simulink model "GFMUPS100k_CPP"  (R2024b)
settings: Solver=ode2  StartTime=0.0  StopTime=6  FixedStep=5e-7  RelTol=1e-3
model workspace (MAT data in the model file):
  amp = 0
  f1 = 1000
undefined symbols (not defined in the file or in its folder): DiscIntNeverNeededParam, L
libraries: spsIGBTDiodeLib x12, slpidlib x12, spsabctodq0Lib x10, spsSeriesRLCBranchLib x9, spsPLL3phLib x8, spsThreePhaseSeriesRLCBranchLib x8, spsDiodeLib x6, dspstat3 x5, spsVoltageMeasurementLib x4, spsThreePhaseVIMeasurementLib x4, spsPower3phInstantaneousLib x3, spsControlledCurrentSourceLib x3
(part 3 of 4)

== system GFMUPS100k_CPP/基于自适应虚拟电流/d轴电压 ==
  presignal : Inport
  Ivd : Inport  Port=2
  MATLAB Function : MATLAB Function  TreatAsAtomicUnit=on
  PID Controller1 : slpidlib/PID Controller  Controller=PI  Form=Parallel  TimeDomain=Discrete-time  UseExternalTs=off  SampleTime=-1  IntegratorMethod=Forward Euler  FilterMethod=Forward Euler  ControllerParametersSource=internal  P=1.4  I=0.2  UseKiTs=off  D=0  UseExternalDerivativeSource=off  N=100  UseFilter=on  TunerSelectOption=Transfer Function Based (PID Tuner App)  InitialConditionSource=internal  InitialConditionForIntegrator=0  InitialConditionForFilter=0  DifferentiatorICPrevScaledInput=0  ExternalReset=none  TrackingMode=off  Kt=1  LimitOutput=off  SatLimitsSource=internal  UpperSaturationLimit=inf  LowerSaturationLimit=-inf  LinearizeAsGain=on  AntiWindupMode=none  Kb=1  LimitIntegrator=off  UpperIntegratorSaturationLimit=inf  LowerIntegratorSaturationLimit=-inf  POutMin=[]  POutMax=[]  IOutMin=[]  IOutMax=[]  DOutMin=[]  DOutMax=[]  NOutMin=[]  NOutMax=[]  SumOutMin=[]  SumOutMax=[]  SaturationOutMin=[]  SaturationOutMax=[]  PParamMin=[]  PParamMax=[]  IParamMin=[]  IParamMax=[]  DParamMin=[]  DParamMax=[]  NParamMin=[]  NParamMax=[]  KbParamMin=[]  KbParamMax=[]  KtParamMin=[]  KtParamMax=[]  KbOutMin=[]  KbOutMax=[]  KtOutMin=[]  KtOutMax=[]  IntegratorOutMin=[]  IntegratorOutMax=[]  FilterOutMin=[]  FilterOutMax=[]  SumI1OutMin=[]  SumI1OutMax=[]  SumI2OutMin=[]  SumI2OutMax=[]  SumI3OutMin=[]  SumI3OutMax=[]  SumI4OutMin=[]  SumI4OutMax=[]  SumDOutMin=[]  SumDOutMax=[]  DifferentiatorOutMin=[]  DifferentiatorOutMax=[]  FilterDiffOutCoefMin=[]  FilterDiffOutCoefMax=[]  ReciprocalOutMin=[]  ReciprocalOutMax=[]  SumDenOutMin=[]  SumDenOutMax=[]  SumNumOutMin=[]  SumNumOutMax=[]  DivideOutMin=[]  DivideOutMax=[]  UdiffTsProdOutMin=[]  UdiffTsProdOutMax=[]  NTsProdOutMin=[]  NTsProdOutMax=[]  UintegralTsProdOutMin=[]  UintegralTsProdOutMax=[]  UngainTsProdOutMin=[]  UngainTsProdOutMax=[]  ClampingZeroOutDataTypeStr=Inherit: Inherit via back propagation  ClampingZeroOutMin=[]  ClampingZeroOutMax=[]  FilterDenConstantOutDataTypeStr=Inherit: Inherit via back propagation  FilterDenConstantOutMin=[]  FilterDenConstantOutMax=[]  PCopyOutDataTypeStr=Inherit: Inherit via back propagation  PCopyOutMin=[]  PCopyOutMax=[]  NCopyOutDataTypeStr=Inherit: Inherit via back propagation  NCopyOutMin=[]  NCopyOutMax=[]  IntegratorContinuousStateAttributes=''  IntegratorStateMustResolveToSignalObject=off  IntegratorRTWStateStorageClass=Auto  FilterContinuousStateAttributes=''  FilterStateMustResolveToSignalObject=off  FilterRTWStateStorageClass=Auto  ParallelPVariant=InternalParameters  IdealPVariant=Disabled  IVariant=InternalParameters  DVariant=Disabled  IntegratorVariant=Discrete  SatVariant=Disabled  AWVariant=Passthrough  PCopyVariant=Disabled  TRVariant=Disabled  FdbkBlocksVariant=Forward  IdealPFdbkVariant=Disabled  SatFdbkVariant=Disabled  DerivativeFilterVariant=Disabled  NVariant=Disabled  NCopyVariant=Disabled_SignalSpec  FilterICVariant=Disabled  IntegratorICVariant=InternalICs  ExternalResetVariant=Disabled  TRSumVariant=Passthrough  SumFdbkVariant=Disabled  SumVariant=Sum_PI  TsampFilterVariant=InternalTs  TsampNgainVariant=Passthrough  TsampIntegralVariant=Disabled_SignalSpec  ExternalSaturationOutDataTypeStr=Inherit: Same as second input  DerivativeSourceVariant=Disabled  PreIntVariant=InternalPreInt
  "deta U " : Outport
  wires:
  MATLAB Function/1(y) -> "deta U "/1
  presignal/1 -> MATLAB Function/2(presignal)
  Ivd/1 -> PID Controller1/1
  PID Controller1/1 -> MATLAB Function/1(u)

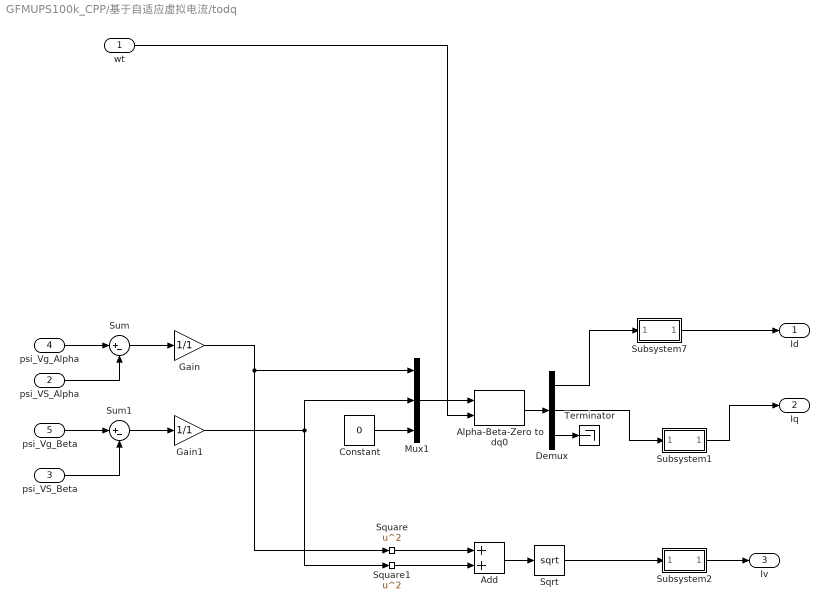
== system GFMUPS100k_CPP/基于自适应虚拟电流/todq ==
  wt : Inport
  psi_VS_Alpha : Inport  Port=2
  psi_VS_Beta : Inport  Port=3
  psi_Vg_Alpha : Inport  Port=4
  psi_Vg_Beta : Inport  Port=5
  Add : Sum
  Alpha-Beta-Zero to dq0 : spsAlphaBetaZerotodq0Lib/Alpha-Beta-Zero to dq0  Alignment=90 degrees behind phase A axis
  Constant : Constant  Value=0
  Demux : Demux  Outputs=3
  Gain : Gain  Gain=1/1
  Gain1 : Gain  Gain=1/1
  Mux1 : Mux  Inputs=3
  Sqrt : Sqrt
  Square : Math  Operator=square
  Square1 : Math  Operator=square
  Subsystem1 : Subsystem
  Subsystem2 : Subsystem
  Subsystem7 : Subsystem
  Sum : Sum  Inputs=|+-
  Sum1 : Sum  Inputs=|+-
  Terminator : Terminator
  Id : Outport
  Iq : Outport  Port=2
  Iv : Outport  Port=3
  wires:
  Demux/2 -> Subsystem1/1(In1)
  Constant/1 -> Mux1/3
  Square/1 -> Add/1
  Add/1 -> Sqrt/1
  Mux1/1 -> Alpha-Beta-Zero to dq0/1
  Square1/1 -> Add/2
  Demux/1 -> Subsystem7/1(In1)
  Gain/1 -> Square/1, Mux1/1
  Sqrt/1 -> Subsystem2/1(In1)
  Demux/3 -> Terminator/1
  Sum1/1 -> Gain1/1
  wt/1 -> Alpha-Beta-Zero to dq0/2
  Sum/1 -> Gain/1
  Alpha-Beta-Zero to dq0/1 -> Demux/1
  Gain1/1 -> Mux1/2, Square1/1
  psi_VS_Beta/1 -> Sum1/2
  psi_Vg_Beta/1 -> Sum1/1
  psi_Vg_Alpha/1 -> Sum/1
  psi_VS_Alpha/1 -> Sum/2
  Subsystem7/1(Out1) -> Id/1
  Subsystem1/1(Out1) -> Iq/1
  Subsystem2/1(Out1) -> Iv/1

== system GFMUPS100k_CPP/基于自适应虚拟电流/标幺 ==
  abc : Inport
  abc1 : Inport  Port=2
  Demux : Demux  Outputs=3
  Demux1 : Demux  Outputs=3
  Gain1 : Gain  Gain=1/311
  Gain2 : Gain  Gain=1/311
  Scope1 : Scope
  Terminator1 : Terminator
  Terminator2 : Terminator
  abc to Alpha-Beta-Zero1 : spsabctoAlphaBetaZeroLib/abc to Alpha-Beta-Zero
  abc to Alpha-Beta-Zero2 : spsabctoAlphaBetaZeroLib/abc to Alpha-Beta-Zero
  Vs_alpha : Outport
  Vs_beta : Outport  Port=2
  Vg_alpha1 : Outport  Port=3
  Vg_beta1 : Outport  Port=4
  wires:
  Demux1/2 -> Vg_beta1/1
  Demux1/3 -> Terminator2/1
  Demux1/1 -> Vg_alpha1/1
  Demux/2 -> Vs_beta/1
  abc to Alpha-Beta-Zero2/1 -> Demux1/1
  abc1/1 -> Gain1/1
  abc to Alpha-Beta-Zero1/1 -> Demux/1
  Demux/3 -> Terminator1/1
  Gain2/1 -> abc to Alpha-Beta-Zero1/1
  Demux/1 -> Vs_alpha/1
  abc/1 -> Gain2/1
  Gain1/1 -> Scope1/1, abc to Alpha-Beta-Zero2/1

== system GFMUPS100k_CPP/基于自适应虚拟电流/自适应PI ==
  Ivq_re : Inport
  Kp_base : Inport  Port=2
  Ki_base : Inport  Port=3
  Gain : Gain
  PID Controller : slpidlib/PID Controller  Controller=PI  Form=Parallel  TimeDomain=Discrete-time  UseExternalTs=off  SampleTime=5e-05  IntegratorMethod=Forward Euler  FilterMethod=Forward Euler  ControllerParametersSource=external  P=1  I=1  UseKiTs=off  D=0  UseExternalDerivativeSource=off  N=100  UseFilter=on  TunerSelectOption=Transfer Function Based (PID Tuner App)  InitialConditionSource=internal  InitialConditionForIntegrator=0  InitialConditionForFilter=0  DifferentiatorICPrevScaledInput=0  ExternalReset=none  TrackingMode=off  Kt=1  LimitOutput=off  SatLimitsSource=internal  UpperSaturationLimit=inf  LowerSaturationLimit=-inf  LinearizeAsGain=on  AntiWindupMode=none  Kb=1  LimitIntegrator=off  UpperIntegratorSaturationLimit=inf  LowerIntegratorSaturationLimit=-inf  POutMin=[]  POutMax=[]  IOutMin=[]  IOutMax=[]  DOutMin=[]  DOutMax=[]  NOutMin=[]  NOutMax=[]  SumOutMin=[]  SumOutMax=[]  SaturationOutMin=[]  SaturationOutMax=[]  PParamMin=[]  PParamMax=[]  IParamMin=[]  IParamMax=[]  DParamMin=[]  DParamMax=[]  NParamMin=[]  NParamMax=[]  KbParamMin=[]  KbParamMax=[]  KtParamMin=[]  KtParamMax=[]  KbOutMin=[]  KbOutMax=[]  KtOutMin=[]  KtOutMax=[]  IntegratorOutMin=[]  IntegratorOutMax=[]  FilterOutMin=[]  FilterOutMax=[]  SumI1OutMin=[]  SumI1OutMax=[]  SumI2OutMin=[]  SumI2OutMax=[]  SumI3OutMin=[]  SumI3OutMax=[]  SumI4OutMin=[]  SumI4OutMax=[]  SumDOutMin=[]  SumDOutMax=[]  DifferentiatorOutMin=[]  DifferentiatorOutMax=[]  FilterDiffOutCoefMin=[]  FilterDiffOutCoefMax=[]  ReciprocalOutMin=[]  ReciprocalOutMax=[]  SumDenOutMin=[]  SumDenOutMax=[]  SumNumOutMin=[]  SumNumOutMax=[]  DivideOutMin=[]  DivideOutMax=[]  UdiffTsProdOutMin=[]  UdiffTsProdOutMax=[]  NTsProdOutMin=[]  NTsProdOutMax=[]  UintegralTsProdOutMin=[]  UintegralTsProdOutMax=[]  UngainTsProdOutMin=[]  UngainTsProdOutMax=[]  ClampingZeroOutDataTypeStr=Inherit: Inherit via back propagation  ClampingZeroOutMin=[]  ClampingZeroOutMax=[]  FilterDenConstantOutDataTypeStr=Inherit: Inherit via back propagation  FilterDenConstantOutMin=[]  FilterDenConstantOutMax=[]  PCopyOutDataTypeStr=Inherit: Inherit via back propagation  PCopyOutMin=[]  PCopyOutMax=[]  NCopyOutDataTypeStr=Inherit: Inherit via back propagation  NCopyOutMin=[]  NCopyOutMax=[]  IntegratorContinuousStateAttributes=''  IntegratorStateMustResolveToSignalObject=off  IntegratorRTWStateStorageClass=Auto  FilterContinuousStateAttributes=''  FilterStateMustResolveToSignalObject=off  FilterRTWStateStorageClass=Auto  ParallelPVariant=ExternalParameters  IdealPVariant=Disabled  IVariant=ExternalParameters  DVariant=Disabled  IntegratorVariant=Discrete  SatVariant=Disabled  AWVariant=Passthrough  PCopyVariant=Disabled  TRVariant=Disabled  FdbkBlocksVariant=Forward  IdealPFdbkVariant=Disabled  SatFdbkVariant=Disabled  DerivativeFilterVariant=Disabled  NVariant=Disabled  NCopyVariant=Disabled_SignalSpec  FilterICVariant=Disabled  IntegratorICVariant=InternalICs  ExternalResetVariant=Disabled  TRSumVariant=Passthrough  SumFdbkVariant=Disabled  SumVariant=Sum_PI  TsampFilterVariant=InternalTs  TsampNgainVariant=Passthrough  TsampIntegralVariant=Disabled_SignalSpec  ExternalSaturationOutDataTypeStr=Inherit: Same as second input  DerivativeSourceVariant=Disabled  PreIntVariant=InternalPreInt
  Scope1 : Scope  NumInputPorts=2
  adaptive_PI : MATLAB Function  TreatAsAtomicUnit=on  SystemSampleTime=5e-05
  预同步 : Subsystem
  预同步1 : Subsystem
  Out1 : Outport
  wires:
  Ki_base/1 -> adaptive_PI/3(Ki_base)
  Ivq_re/1 -> adaptive_PI/1(Ivq_re), PID Controller/1
  adaptive_PI/1(Kp_act) -> 预同步/1(d_theta)
  Kp_base/1 -> adaptive_PI/2(Kp_base)
  adaptive_PI/2(Ki_act) -> 预同步1/1(d_theta)
  Gain/1 -> Out1/1
  PID Controller/1 -> Gain/1
  预同步/1(Out1) -> PID Controller/2, Scope1/1
  预同步1/1(Out1) -> PID Controller/3, Scope1/2

== system GFMUPS100k_CPP/基于转dq的预同步控制1/电压预同步 ==
  Vg : Inport
  Vabc : Inport  Port=2
  presignal : Inport  Port=3
  Constant1 : Constant  Value=0
  PID Controller2 : slpidlib/PID Controller  Controller=PI  Form=Parallel  TimeDomain=Discrete-time  UseExternalTs=off  SampleTime=5e-05  IntegratorMethod=Forward Euler  FilterMethod=Forward Euler  ControllerParametersSource=internal  P=0.8  I=0  UseKiTs=off  D=0  UseExternalDerivativeSource=off  N=100  UseFilter=on  TunerSelectOption=Transfer Function Based (PID Tuner App)  InitialConditionSource=internal  InitialConditionForIntegrator=0  InitialConditionForFilter=0  DifferentiatorICPrevScaledInput=0  ExternalReset=none  TrackingMode=off  Kt=1  LimitOutput=off  SatLimitsSource=internal  UpperSaturationLimit=inf  LowerSaturationLimit=-inf  LinearizeAsGain=on  AntiWindupMode=none  Kb=1  LimitIntegrator=off  UpperIntegratorSaturationLimit=inf  LowerIntegratorSaturationLimit=-inf  POutMin=[]  POutMax=[]  IOutMin=[]  IOutMax=[]  DOutMin=[]  DOutMax=[]  NOutMin=[]  NOutMax=[]  SumOutMin=[]  SumOutMax=[]  SaturationOutMin=[]  SaturationOutMax=[]  PParamMin=[]  PParamMax=[]  IParamMin=[]  IParamMax=[]  DParamMin=[]  DParamMax=[]  NParamMin=[]  NParamMax=[]  KbParamMin=[]  KbParamMax=[]  KtParamMin=[]  KtParamMax=[]  KbOutMin=[]  KbOutMax=[]  KtOutMin=[]  KtOutMax=[]  IntegratorOutMin=[]  IntegratorOutMax=[]  FilterOutMin=[]  FilterOutMax=[]  SumI1OutMin=[]  SumI1OutMax=[]  SumI2OutMin=[]  SumI2OutMax=[]  SumI3OutMin=[]  SumI3OutMax=[]  SumI4OutMin=[]  SumI4OutMax=[]  SumDOutMin=[]  SumDOutMax=[]  DifferentiatorOutMin=[]  DifferentiatorOutMax=[]  FilterDiffOutCoefMin=[]  FilterDiffOutCoefMax=[]  ReciprocalOutMin=[]  ReciprocalOutMax=[]  SumDenOutMin=[]  SumDenOutMax=[]  SumNumOutMin=[]  SumNumOutMax=[]  DivideOutMin=[]  DivideOutMax=[]  UdiffTsProdOutMin=[]  UdiffTsProdOutMax=[]  NTsProdOutMin=[]  NTsProdOutMax=[]  UintegralTsProdOutMin=[]  UintegralTsProdOutMax=[]  UngainTsProdOutMin=[]  UngainTsProdOutMax=[]  ClampingZeroOutDataTypeStr=Inherit: Inherit via back propagation  ClampingZeroOutMin=[]  ClampingZeroOutMax=[]  FilterDenConstantOutDataTypeStr=Inherit: Inherit via back propagation  FilterDenConstantOutMin=[]  FilterDenConstantOutMax=[]  PCopyOutDataTypeStr=Inherit: Inherit via back propagation  PCopyOutMin=[]  PCopyOutMax=[]  NCopyOutDataTypeStr=Inherit: Inherit via back propagation  NCopyOutMin=[]  NCopyOutMax=[]  IntegratorContinuousStateAttributes=''  IntegratorStateMustResolveToSignalObject=off  IntegratorRTWStateStorageClass=Auto  FilterContinuousStateAttributes=''  FilterStateMustResolveToSignalObject=off  FilterRTWStateStorageClass=Auto  ParallelPVariant=InternalParameters  IdealPVariant=Disabled  IVariant=InternalParameters  DVariant=Disabled  IntegratorVariant=Discrete  SatVariant=Disabled  AWVariant=Passthrough  PCopyVariant=Disabled  TRVariant=Disabled  FdbkBlocksVariant=Forward  IdealPFdbkVariant=Disabled  SatFdbkVariant=Disabled  DerivativeFilterVariant=Disabled  NVariant=Disabled  NCopyVariant=Disabled_SignalSpec  FilterICVariant=Disabled  IntegratorICVariant=InternalICs  ExternalResetVariant=Disabled  TRSumVariant=Passthrough  SumFdbkVariant=Disabled  SumVariant=Sum_PI  TsampFilterVariant=InternalTs  TsampNgainVariant=Passthrough  TsampIntegralVariant=Disabled_SignalSpec  ExternalSaturationOutDataTypeStr=Inherit: Same as second input  DerivativeSourceVariant=Disabled  PreIntVariant=InternalPreInt
  RMS1 : dspstat3/RMS  run=off  directionMode=Each column  dimension=1  InputProcessing=Columns as channels (frame based)  reset_popup=None
  RMS2 : dspstat3/RMS  run=off  directionMode=Each column  dimension=1  InputProcessing=Columns as channels (frame based)  reset_popup=None
  Scope : Scope
  Sum4 : Sum  Inputs=|+-
  Switch : Switch  Criteria=u2 > Threshold  SaturateOnIntegerOverflow=off  InputSameDT=off
  d_U : Outport
  wires:
  presignal/1 -> Switch/2
  Constant1/1 -> Switch/3
  PID Controller2/1 -> Switch/1
  Sum4/1 -> Scope/1, PID Controller2/1
  Switch/1 -> d_U/1
  Vg/1 -> RMS2/1
  Vabc/1 -> RMS1/1
  RMS2/1 -> Sum4/1
  RMS1/1 -> Sum4/2

== system GFMUPS100k_CPP/基于转dq的预同步控制1/相位预同步 ==
  Vg : Inport
  Vabc : Inport  Port=2
  presignal : Inport  Port=3
  Constant5 : Constant  Value=0
  Demux : Demux  Outputs=3
  Gain : Gain  Gain=-1
  PID Controller1 : slpidlib/PID Controller  Controller=PI  Form=Parallel  TimeDomain=Discrete-time  UseExternalTs=off  SampleTime=5e-05  IntegratorMethod=Forward Euler  FilterMethod=Forward Euler  ControllerParametersSource=internal  P=0.4  I=0.01  UseKiTs=off  D=0  UseExternalDerivativeSource=off  N=100  UseFilter=on  TunerSelectOption=Transfer Function Based (PID Tuner App)  InitialConditionSource=internal  InitialConditionForIntegrator=0  InitialConditionForFilter=0  DifferentiatorICPrevScaledInput=0  ExternalReset=none  TrackingMode=off  Kt=1  LimitOutput=off  SatLimitsSource=internal  UpperSaturationLimit=inf  LowerSaturationLimit=-inf  LinearizeAsGain=on  AntiWindupMode=none  Kb=1  LimitIntegrator=off  UpperIntegratorSaturationLimit=inf  LowerIntegratorSaturationLimit=-inf  POutMin=[]  POutMax=[]  IOutMin=[]  IOutMax=[]  DOutMin=[]  DOutMax=[]  NOutMin=[]  NOutMax=[]  SumOutMin=[]  SumOutMax=[]  SaturationOutMin=[]  SaturationOutMax=[]  PParamMin=[]  PParamMax=[]  IParamMin=[]  IParamMax=[]  DParamMin=[]  DParamMax=[]  NParamMin=[]  NParamMax=[]  KbParamMin=[]  KbParamMax=[]  KtParamMin=[]  KtParamMax=[]  KbOutMin=[]  KbOutMax=[]  KtOutMin=[]  KtOutMax=[]  IntegratorOutMin=[]  IntegratorOutMax=[]  FilterOutMin=[]  FilterOutMax=[]  SumI1OutMin=[]  SumI1OutMax=[]  SumI2OutMin=[]  SumI2OutMax=[]  SumI3OutMin=[]  SumI3OutMax=[]  SumI4OutMin=[]  SumI4OutMax=[]  SumDOutMin=[]  SumDOutMax=[]  DifferentiatorOutMin=[]  DifferentiatorOutMax=[]  FilterDiffOutCoefMin=[]  FilterDiffOutCoefMax=[]  ReciprocalOutMin=[]  ReciprocalOutMax=[]  SumDenOutMin=[]  SumDenOutMax=[]  SumNumOutMin=[]  SumNumOutMax=[]  DivideOutMin=[]  DivideOutMax=[]  UdiffTsProdOutMin=[]  UdiffTsProdOutMax=[]  NTsProdOutMin=[]  NTsProdOutMax=[]  UintegralTsProdOutMin=[]  UintegralTsProdOutMax=[]  UngainTsProdOutMin=[]  UngainTsProdOutMax=[]  ClampingZeroOutDataTypeStr=Inherit: Inherit via back propagation  ClampingZeroOutMin=[]  ClampingZeroOutMax=[]  FilterDenConstantOutDataTypeStr=Inherit: Inherit via back propagation  FilterDenConstantOutMin=[]  FilterDenConstantOutMax=[]  PCopyOutDataTypeStr=Inherit: Inherit via back propagation  PCopyOutMin=[]  PCopyOutMax=[]  NCopyOutDataTypeStr=Inherit: Inherit via back propagation  NCopyOutMin=[]  NCopyOutMax=[]  IntegratorContinuousStateAttributes=''  IntegratorStateMustResolveToSignalObject=off  IntegratorRTWStateStorageClass=Auto  FilterContinuousStateAttributes=''  FilterStateMustResolveToSignalObject=off  FilterRTWStateStorageClass=Auto  ParallelPVariant=InternalParameters  IdealPVariant=Disabled  IVariant=InternalParameters  DVariant=Disabled  IntegratorVariant=Discrete  SatVariant=Disabled  AWVariant=Passthrough  PCopyVariant=Disabled  TRVariant=Disabled  FdbkBlocksVariant=Forward  IdealPFdbkVariant=Disabled  SatFdbkVariant=Disabled  DerivativeFilterVariant=Disabled  NVariant=Disabled  NCopyVariant=Disabled_SignalSpec  FilterICVariant=Disabled  IntegratorICVariant=InternalICs  ExternalResetVariant=Disabled  TRSumVariant=Passthrough  SumFdbkVariant=Disabled  SumVariant=Sum_PI  TsampFilterVariant=InternalTs  TsampNgainVariant=Passthrough  TsampIntegralVariant=Disabled_SignalSpec  ExternalSaturationOutDataTypeStr=Inherit: Same as second input  DerivativeSourceVariant=Disabled  PreIntVariant=InternalPreInt
  PLL (3ph) : spsPLL3phLib/PLL (3ph)  Fmin=45  Par_Init=[0, 60]  ParK=[180, 3200, 1]  TcD=1e-4  MaxRateChangeFreq=12  FilterCutOffFreq=25  Ts=0  AGC=on
  Scope : Scope
  Scope1 : Scope
  Switch : Switch  Criteria=u2 > Threshold  SaturateOnIntegerOverflow=off  InputSameDT=off
  Terminator : Terminator
  Terminator1 : Terminator
  Terminator2 : Terminator
  abc to dq0 : spsabctodq0Lib/abc to dq0  Alignment=90 degrees behind phase A axis
  c_theta : Outport
  wires:
  Constant5/1 -> Switch/3
  PID Controller1/1 -> Switch/1
  Switch/1 -> Scope1/1, c_theta/1
  presignal/1 -> Switch/2
  Vg/1 -> PLL (3ph)/1
  Vabc/1 -> abc to dq0/1
  abc to dq0/1 -> Demux/1
  PLL (3ph)/2 -> abc to dq0/2
  PLL (3ph)/1 -> Terminator/1
  Demux/3 -> Terminator2/1
  Demux/1 -> Terminator1/1
  Demux/2 -> Gain/1
  Gain/1 -> Scope/1, PID Controller1/1

== system GFMUPS100k_CPP/相角差计算/Subsystem1 ==
  abc : Inport
  abc1 : Inport  Port=2
  Add : Sum  Inputs=+-
  PLL (3ph)1 : spsPLL3phLib/PLL (3ph)  Fmin=45  Par_Init=[0, 60]  ParK=[180, 3200, 1]  TcD=1e-4  MaxRateChangeFreq=12  FilterCutOffFreq=25  Ts=0  AGC=on
  PLL (3ph)2 : spsPLL3phLib/PLL (3ph)  Fmin=45  Par_Init=[0, 60]  ParK=[180, 3200, 1]  TcD=1e-4  MaxRateChangeFreq=12  FilterCutOffFreq=25  Ts=0  AGC=on
  Terminator8 : Terminator
  Terminator9 : Terminator
  Out1 : Outport
  wires:
  PLL (3ph)1/1 -> Terminator9/1
  PLL (3ph)2/2 -> Add/1
  PLL (3ph)2/1 -> Terminator8/1
  PLL (3ph)1/2 -> Add/2
  Add/1 -> Out1/1
  abc/1 -> PLL (3ph)2/1
  abc1/1 -> PLL (3ph)1/1

== system GFMUPS100k_CPP/相角差计算/Subsystem2 ==
  In1 : Inport
  Add : Sum  Inputs=+-
  Add4 : Sum
  Constant : Constant  Value=2*pi
  Constant1 : Constant  Value=pi
  Constant2 : Constant  Value=pi
  Mod : Math  Operator=mod
  dete_theta : Outport
  wires:
  In1/1 -> Add4/1
  Constant1/1 -> Add/2
  Add4/1 -> Mod/1
  Constant/1 -> Mod/2
  Mod/1 -> Add/1
  Constant2/1 -> Add4/2
  Add/1 -> dete_theta/1

== system GFMUPS100k_CPP/VSG_Control/无功控制环1/Subsystem1 ==
  In1 : Inport
  Discrete-Time Integrator : DiscreteIntegrator  SampleTime=1/20000  ICPrevOutput=DiscIntNeverNeededParam  ICPrevScaledInput=DiscIntNeverNeededParam
  Gain1 : Gain  Gain=2*pi*50
  Gain2 : Gain
  Sum3 : Sum  Inputs=|+-
  Out1 : Outport
  wires:
  Sum3/1 -> Gain1/1
  Gain1/1 -> Discrete-Time Integrator/1
  Gain2/1 -> Sum3/2
  In1/1 -> Sum3/1
  Discrete-Time Integrator/1 -> Gain2/1, Out1/1

== system GFMUPS100k_CPP/VSG_Control/无功控制环1/Subsystem2 ==
  In1 : Inport
  Discrete-Time Integrator : DiscreteIntegrator  SampleTime=1/20000  ICPrevOutput=DiscIntNeverNeededParam  ICPrevScaledInput=DiscIntNeverNeededParam
  Gain1 : Gain  Gain=2*pi*50
  Gain2 : Gain
  Sum3 : Sum  Inputs=|+-
  Out1 : Outport
  wires:
  Discrete-Time Integrator/1 -> Out1/1, Gain2/1
  In1/1 -> Sum3/1
  Gain2/1 -> Sum3/2
  Gain1/1 -> Discrete-Time Integrator/1
  Sum3/1 -> Gain1/1

== system GFMUPS100k_CPP/VSG_Control/有功控制环/预同步 ==
  d_theta : Inport
  Discrete-Time Integrator : DiscreteIntegrator  SampleTime=5e-05  ICPrevOutput=DiscIntNeverNeededParam  ICPrevScaledInput=DiscIntNeverNeededParam
  Gain1 : Gain  Gain=1/0.03
  Gain2 : Gain
  Saturation : Saturate  Commented=on  UpperLimit=401.23  LowerLimit=-9.54
  Scope : Scope  NumInputPorts=2
  Sum3 : Sum  Inputs=|+-
  Out1 : Outport
  wires:
  Discrete-Time Integrator/1 -> Scope/2, Out1/1, Gain2/1
  Gain1/1 -> Discrete-Time Integrator/1
  Sum3/1 -> Gain1/1
  Gain2/1 -> Sum3/2
  d_theta/1 -> Scope/1, Sum3/1

== system GFMUPS100k_CPP/VSG_Control/虚拟阻抗（scr补偿）/Subsystem1 ==
  In1 : Inport
  Discrete-Time Integrator : DiscreteIntegrator  SampleTime=1/20000  ICPrevOutput=DiscIntNeverNeededParam  ICPrevScaledInput=DiscIntNeverNeededParam
  Gain1 : Gain  Gain=2*pi*500
  Gain2 : Gain
  Sum3 : Sum  Inputs=|+-
  Out1 : Outport
  wires:
  Discrete-Time Integrator/1 -> Out1/1, Gain2/1
  In1/1 -> Sum3/1
  Gain2/1 -> Sum3/2
  Gain1/1 -> Discrete-Time Integrator/1
  Sum3/1 -> Gain1/1

== system GFMUPS100k_CPP/VSG_Control/虚拟阻抗（scr补偿）/Subsystem7 ==
  In1 : Inport
  Discrete-Time Integrator : DiscreteIntegrator  SampleTime=1/20000  ICPrevOutput=DiscIntNeverNeededParam  ICPrevScaledInput=DiscIntNeverNeededParam
  Gain1 : Gain  Gain=2*pi*500
  Gain2 : Gain
  Sum3 : Sum  Inputs=|+-
  Out1 : Outport
  wires:
  Sum3/1 -> Gain1/1
  Gain1/1 -> Discrete-Time Integrator/1
  Gain2/1 -> Sum3/2
  In1/1 -> Sum3/1
  Discrete-Time Integrator/1 -> Gain2/1, Out1/1

== system GFMUPS100k_CPP/基于自适应虚拟电流/todq/Subsystem1 ==
  In1 : Inport
  Discrete-Time Integrator : DiscreteIntegrator  SampleTime=1/20000  ICPrevOutput=DiscIntNeverNeededParam  ICPrevScaledInput=DiscIntNeverNeededParam
  Gain1 : Gain  Gain=2*pi*50
  Gain2 : Gain
  Sum3 : Sum  Inputs=|+-
  Out1 : Outport
  wires:
  Discrete-Time Integrator/1 -> Out1/1, Gain2/1
  In1/1 -> Sum3/1
  Gain2/1 -> Sum3/2
  Gain1/1 -> Discrete-Time Integrator/1
  Sum3/1 -> Gain1/1

== system GFMUPS100k_CPP/基于自适应虚拟电流/todq/Subsystem2 ==
  In1 : Inport
  Discrete-Time Integrator : DiscreteIntegrator  SampleTime=1/20000  ICPrevOutput=DiscIntNeverNeededParam  ICPrevScaledInput=DiscIntNeverNeededParam
  Gain1 : Gain  Gain=2*pi*50
  Gain2 : Gain
  Sum3 : Sum  Inputs=|+-
  Out1 : Outport
  wires:
  Sum3/1 -> Gain1/1
  Gain1/1 -> Discrete-Time Integrator/1
  Gain2/1 -> Sum3/2
  In1/1 -> Sum3/1
  Discrete-Time Integrator/1 -> Gain2/1, Out1/1

== system GFMUPS100k_CPP/基于自适应虚拟电流/todq/Subsystem7 ==
  In1 : Inport
  Discrete-Time Integrator : DiscreteIntegrator  SampleTime=1/20000  ICPrevOutput=DiscIntNeverNeededParam  ICPrevScaledInput=DiscIntNeverNeededParam
  Gain1 : Gain  Gain=2*pi*50
  Gain2 : Gain
  Sum3 : Sum  Inputs=|+-
  Out1 : Outport
  wires:
  Sum3/1 -> Gain1/1
  Gain1/1 -> Discrete-Time Integrator/1
  Gain2/1 -> Sum3/2
  In1/1 -> Sum3/1
  Discrete-Time Integrator/1 -> Gain2/1, Out1/1

== system GFMUPS100k_CPP/基于自适应虚拟电流/自适应PI/预同步 ==
  d_theta : Inport
  Discrete-Time Integrator : DiscreteIntegrator  SampleTime=5e-05  ICPrevOutput=DiscIntNeverNeededParam  ICPrevScaledInput=DiscIntNeverNeededParam
  Gain1 : Gain  Gain=1/0.03
  Gain2 : Gain
  Saturation : Saturate  Commented=on  UpperLimit=401.23  LowerLimit=-9.54
  Sum3 : Sum  Inputs=|+-
  Out1 : Outport
  wires:
  Discrete-Time Integrator/1 -> Out1/1, Gain2/1
  Gain1/1 -> Discrete-Time Integrator/1
  Sum3/1 -> Gain1/1
  Gain2/1 -> Sum3/2
  d_theta/1 -> Sum3/1

== system GFMUPS100k_CPP/基于自适应虚拟电流/自适应PI/预同步1 ==
  d_theta : Inport
  Discrete-Time Integrator : DiscreteIntegrator  SampleTime=5e-05  ICPrevOutput=DiscIntNeverNeededParam  ICPrevScaledInput=DiscIntNeverNeededParam
  Gain1 : Gain  Gain=1/0.03
  Gain2 : Gain
  Saturation : Saturate  Commented=on  UpperLimit=401.23  LowerLimit=-9.54
  Sum3 : Sum  Inputs=|+-
  Out1 : Outport
  wires:
  d_theta/1 -> Sum3/1
  Gain2/1 -> Sum3/2
  Sum3/1 -> Gain1/1
  Gain1/1 -> Discrete-Time Integrator/1
  Discrete-Time Integrator/1 -> Gain2/1, Out1/1

== matlab function GFMUPS100k_CPP/SVPWM调制/SVPWM/第一大扇区羊角波分配 ==
  data: n input; T1 input; T2 input; T3 input; t11 output; t21 output; t31 output
function [t11,t21,t31] = vectorshare(n,T1,T2,T3)
t11=0;
t21=0;
t31=0;
if(n==1)
    t11=T1/2;
    t21=-T1/2;
    t31=-T1/2-T2;
end
if(n==2)
    t11=T1/2+T3;
    t21=T1/2;
    t31=-T1/2;
end
if(n==3)
    t11=T1/2+T3;
    t21=-T1/2;
    t31=-T1/2-T2-T3;
end
if(n==4)
    t11=T1/2+T2+T3;
    t21=T1/2;
    t31=-T1/2-T2;
end
if(n==5)
    t11=T1/2+T2+T3;
    t21=-T1/2-T2;
    t31=-T1/2-T2-T3;
end
if(n==6)
    t11=T1/2+T2+T3;
    t21=T1/2+T3;
    t31=-T1/2-T2-T3;
end

== matlab function GFMUPS100k_CPP/SVPWM调制/SVPWM/第二大扇区羊角波分配 ==
  data: n input; T1 input; T2 input; T3 input; t11 output; t21 output; t31 output
function [t11,t21,t31] = switchshare(n,T1,T2,T3)
t11=0;
t21=0;
t31=0;
if(n==1)
    t11=T1/2;
    t21=T1/2+T3;
    t31=-T1/2;
end
if(n==2)
    t11=-T1/2;
    t21=T1/2;
    t31=-T1/2-T2;
end
if(n==3)
    t11=T1/2;
    t21=T1/2+T2+T3;
    t31=-T1/2-T2;
end
if(n==4)
    t11=-T1/2;
    t21=T1/2+T3;
    t31=-T1/2-T2-T3;
end
if(n==5)
    t11=T1/2+T3;
    t21=T1/2+T2+T3;
    t31=-T1/2-T2-T3;
end
if(n==6)
    t11=-T1/2-T2;
    t21=T1/2+T3+T2;
    t31=-T1/2-T2-T3;
end

== matlab function GFMUPS100k_CPP/SVPWM调制/SVPWM/羊角波生成 ==
  data: N input; t11 input; t12 input; t13 input; YJA output; YJB output; YJC output; t21 input; t22 input; t23 input
function [YJA,YJB,YJC] = vectorshare(N,t11,t12,t13,t21,t22,t23)
YJA=0;
YJB=0;
YJC=0;
if(N==1)
    YJA=t11;
    YJB=t12;
    YJC=t13;
end
if(N==2)
    YJA=t21;
    YJB=t22;
    YJC=t23;
end
if(N==3)
    YJA=t13;
    YJB=t11;
    YJC=t12;
end
if(N==4)
    YJA=t23;
    YJB=t21;
    YJC=t22;
end
if(N==5)
    YJA=t12;
    YJB=t13;
    YJC=t11;
end
if(N==6)
    YJA=t22;
    YJB=t23;
    YJC=t21;
end

== matlab function GFMUPS100k_CPP/基于自适应虚拟电流/MATLAB Function ==
  data: u input; y output; presignal input
function y = fcn(u, presignal)
    % 如果 presignal 大于 0，输出 y 等于 u
    % 否则输出 y 等于 0
    if presignal > 0
        y = u;
    else
        y = 0;
    end
end

== matlab function GFMUPS100k_CPP/基于自适应虚拟电流/d轴电压/MATLAB Function ==
  data: u input; y output; presignal input
function y = fcn(u, presignal)
    % 如果 presignal 大于 0，输出 y 等于 u
    % 否则输出 y 等于 0
    if presignal > 0
        y = u;
    else
        y = 0;
    end
end

== matlab function GFMUPS100k_CPP/Grid_Impedance_Estimator/Positive_Sequence ==
  data: vabc input; E output; iuabc input; ilabc input; t input; reset input; source input; Vg output; theta output; Pu output; Qu output; PL output; QL output; ready output
function [E,Vg,theta,Pu,Qu,PL,QL,ready] = positive_sequence_inputs(vabc,iuabc,ilabc,t,reset,source)
%#codegen
% 200 samples at 100 us = one 50-Hz cycle, fixed-size positive sequence DFT.
% source = [line-line RMS volts, Hz, phase A sine angle in degrees].
persistent buffer sums index count
if isempty(count)   %200个采样点， 采样周期为1e-4，200*Ts，刚好是一个完整的50HZ周期  Sum保存200个点的累加  count表示收集了多少有效采样点
    buffer = zeros(6,200); sums = zeros(6,1); index = 1; count = 0;
end
if reset ~= 0
    buffer(:) = 0; sums(:) = 0; index = 1; count = 0;
end
E=0; Vg=source(1)*sqrt(2/3); theta=0;
Pu=0; Qu=0; PL=0; QL=0; ready=false;
if ~all(isfinite([vabc(:);iuabc(:);ilabc(:);t]))  %检查是不是所有输入都是正常有限数值
    buffer(:)=0; sums(:)=0; index=1; count=0;
    return
end
phi = 2*pi*source(2)*t + source(3)*pi/180-pi/2;  %电网参考角
c=cos(phi); s=sin(phi);
va=(2*vabc(1)-vabc(2)-vabc(3))/3;%abc转到β轴
vb=(vabc(2)-vabc(3))/sqrt(3);
ua=(2*iuabc(1)-iuabc(2)-iuabc(3))/3;
ub=(iuabc(2)-iuabc(3))/sqrt(3);
la=(2*ilabc(1)-ilabc(2)-ilabc(3))/3;
lb=(ilabc(2)-ilabc(3))/sqrt(3);
sample=[va*c+vb*s;vb*c-va*s;ua*c+ub*s;ub*c-ua*s;la*c+lb*s;lb*c-la*s];
sums=sums-buffer(:,index)+sample;%把200个点中旧的数据删除，加入新的数据
buffer(:,index)=sample;
index=index+1;
if index>200, index=1; end
count=min(count+1,200);
v=sums/200;   %在不足200点的时候也除以200，所以在200个点前数据会偏小  ready的作用就是其=1时才使用这些数据
E=hypot(v(1),v(2)); theta=atan2(v(2),v(1));%计算幅值和相角差
Pu=1.5*(v(1)*v(3)+v(2)*v(4));
Qu=1.5*(v(2)*v(3)-v(1)*v(4));
PL=1.5*(v(1)*v(5)+v(2)*v(6));
QL=1.5*(v(2)*v(5)-v(1)*v(6));
ready=count>=200 && reset==0;
end

== matlab function GFMUPS100k_CPP/Grid_Impedance_Estimator/Newton_Estimator ==
  data: E input; Rg_hat output; Vg input; theta input; Pu input; Qu input; PL input; QL input; enable input; reset input; cfg input; Xg_hat output; Lg_hat output; Pg output; Qg output; f1 output; f2 output; detJ output; iterNum output; converged output; valid output
function [Rg_hat,Xg_hat,Lg_hat,Pg,Qg,f1,f2,detJ,iterNum,converged,valid] = grid_impedance_estimator(E,Vg,theta,Pu,Qu,PL,QL,enable,reset,cfg)
%#codegen
% cfg = [Rg0 Xg0 alpha eta Pmin Qmin dVmin thetaMin Emin sensitivityMin]
% E,Vg: positive-sequence PHASE PEAK volts; theta: PCC minus grid radians.
% Pu/Qu: UPS into PCC; PL/QL: PCC into load; all powers are signed W/var.
persistent Rg_last Xg_last Pbar Qbar initialized
if isempty(initialized)
    Rg_last = min(max(cfg(1),0.001),10);   %给牛顿法设置初值
    Xg_last = min(max(cfg(2),0.001),10);
    Pbar = 0; Qbar = 0; initialized = false;
end
Pg = Pu-PL; Qg = Qu-QL;
f1 = 0; f2 = 0; detJ = 0; iterNum = 0;
converged = false; valid = false;
if reset ~= 0
    Rg_last = min(max(cfg(1),0.001),10);
    Xg_last = min(max(cfg(2),0.001),10);
    Pbar = 0; Qbar = 0; initialized = false;
end
Rg_hat = Rg_last; Xg_hat = Xg_last;
Lg_hat = Xg_hat/(2*pi*50);
if reset ~= 0 || enable == 0
    return
end
if ~all(isfinite([E Vg theta Pu Qu PL QL])) || E < cfg(9) || Vg < cfg(9)
    return
end
if ~initialized
    Pbar = Pg; Qbar = Qg; initialized = true;
else
    Pbar = (1-cfg(3))*Pbar + cfg(3)*Pg;  %低通滤波
    Qbar = (1-cfg(3))*Qbar + cfg(3)*Qg;
end
theta = atan2(sin(theta),cos(theta));
A = E*E-Vg*E*cos(theta);
B = Vg*E*sin(theta);
[f1,f2,J,detJ] = residual(Rg_last,Xg_last,A,B,Pbar,Qbar);
lowSignals = abs(Pg)<cfg(5) && abs(Qg)<cfg(6) && ...     %认定激励太小，无法进行迭代
    abs(E-Vg)<cfg(7) && abs(theta)<cfg(8);
% Both Jacobian singular values equal 1.5*hypot(A,B)/(R^2+X^2).
sensitivity = 1.5*hypot(A,B)/(Rg_last^2+Xg_last^2);        %判断P Q对R和X变化的敏感性
if lowSignals || sensitivity < cfg(10)
    return
end
R = Rg_last; X = Xg_last;
for k = 1:10
    [f1,f2,J,detJ] = residual(R,X,A,B,Pbar,Qbar);
    if abs(f1)<1e-4 && abs(f2)<1e-4
        converged = true;
        break
    end
    if ~all(isfinite([f1 f2 detJ J(1,:) J(2,:)]))
        break
    end
    if abs(detJ)<1e-10   %改为梯度下降算法 当奇异值接近奇异时
        grad_R = f1*J(1,1)+f2*J(2,1);
        grad_X = f1*J(1,2)+f2*J(2,2);
        step = -cfg(4)*[grad_R;grad_X];
    else
        step = -(J\[f1;f2]);
    end
    if ~all(isfinite(step))
        break
    end
    step = min(max(step,-0.1),0.1);
    R = min(max(R+step(1),0.001),10);
    X = min(max(X+step(2),0.001),10);
    iterNum = k;
end
% Check the result of update 10 as well as earlier iterates.
[f1,f2,J,detJ] = residual(R,X,A,B,Pbar,Qbar);
converged = isfinite(f1) && isfinite(f2) && abs(f1)<1e-4 && abs(f2)<1e-4;
if converged
    Rg_last = R; Xg_last = X; valid = true;
end
Rg_hat = Rg_last; Xg_hat = Xg_last;
Lg_hat = Xg_hat/(2*pi*50);
% Diagnostics always describe the emitted (possibly held) estimate.
[f1,f2,J,detJ] = residual(Rg_hat,Xg_hat,A,B,Pbar,Qbar);
end

function [f1,f2,J,detJ] = residual(R,X,A,B,P,Q)
D = R*R+X*X;
U = R*A+X*B; V = X*A-R*B;
f1 = P-1.5*U/D;
f2 = Q-1.5*V/D;
j11 = 1.5*(2*R*U-A*D)/(D*D);
j12 = 1.5*(2*X*U-B*D)/(D*D);
j21 = 1.5*(2*R*V+B*D)/(D*D);
j22 = 1.5*(2*X*V-A*D)/(D*D);
J = [j11 j12;j21 j22];
detJ = det(J);
end

== matlab function GFMUPS100k_CPP/Operating_Point_Estimator ==
  data: E input; E0 output; theta input; Vg input; Pg input; Qg input; enable input; reset input; cfg input; theta0 output; Vg0 output; Pg0 output; Qg0 output; steady output; locked output; Ebar output; thetabar output; Vgbar output; Pgbar output; Qgbar output
function [E0,theta0,Vg0,Pg0,Qg0,...
          steady,locked,...
          Ebar,thetabar,Vgbar,Pgbar,Qgbar] = ...
          steady_point_estimator(E,theta,Vg,Pg,Qg,enable,reset,cfg)
%#codegen
%
% 稳态工作点提取器
%
% 基本思想：
% 1. 按参考论文采用递推平均滤波：
%       x_bar(k) = (1-alpha)*x_bar(k-1) + alpha*x(k)
%
% 2. 根据滤波后变量变化速率判断系统是否进入准稳态。
%
% 3. 连续满足稳态条件 holdTime 后，
%    锁存 E0、theta0、Vg0、Pg0、Qg0。
%
% ------------------------- 输入 -------------------------
% E      : PCC正序电压幅值
% theta  : PCC相对于电网的功角 [rad]
%          theta = angle(Upcc+) - angle(Vg+)
% Vg     : 电网正序电压幅值
% Pg     : PCC -> 电网支路有功功率 [W]
% Qg     : PCC -> 电网支路无功功率 [var]
% enable : 1=运行工作点估计器
% reset  : 1=清除原工作点并重新寻找
%
% cfg = [alpha, Ts, ...
%        rE_max, rTheta_max, rVg_max, ...
%        rP_max, rQ_max, ...
%        holdTime, updateMode]
%
% alpha       : 递推平均遗忘因子，0<alpha<=1
% Ts          : 本函数执行采样时间 [s]
% rE_max      : |dEbar/dt|允许最大值 [V/s]
% rTheta_max  : |dtheta_bar/dt|最大值 [rad/s]
% rVg_max     : |dVgbar/dt|最大值 [V/s]
% rP_max      : |dPgbar/dt|最大值 [W/s]
% rQ_max      : |dQgbar/dt|最大值 [var/s]
% holdTime    : 连续满足稳态条件的时间 [s]
% updateMode  : 0 = 只锁存第一次稳态点
%               1 = 每次经历扰动并重新稳定后更新工作点
%
% ------------------------- 输出 -------------------------
% E0,theta0,Vg0,Pg0,Qg0 : 锁存的稳态工作点
% steady                : 当前是否满足稳态条件
% locked                : 是否已经获得有效工作点
% Ebar,...              : 滤波后的实时变量
%
% 注意：
% 用于参考论文式(3)-(5)时，E、Vg的幅值定义必须与论文一致。

persistent E_f theta_f Vg_f P_f Q_f
persistent E0_z theta0_z Vg0_z P0_z Q0_z
persistent stableCount
persistent locked_z
persistent prevSteady
persistent initialized

%% 参数读取
alpha      = cfg(1);
Ts         = cfg(2);
rE_max     = cfg(3);
rTheta_max = cfg(4);
rVg_max    = cfg(5);
rP_max     = cfg(6);
rQ_max     = cfg(7);
holdTime   = cfg(8);
updateMode = cfg(9);

% 基本保护
alpha = min(max(alpha,1e-6),1);

if Ts <= 0
    Ts = 1e-4;
end

Nhold = max(1,ceil(holdTime/Ts));   %ceil向上取整数

%% 初始化
if isempty(initialized)
    E_f     = E;
    theta_f = wrapToPiLocal(theta);
    Vg_f    = Vg;
    P_f     = Pg;
    Q_f     = Qg;

    E0_z     = E;
    theta0_z = wrapToPiLocal(theta);
    Vg0_z    = Vg;
    P0_z     = Pg;
    Q0_z     = Qg;

    stableCount = 0;
    locked_z    = false;
    prevSteady  = false;
    initialized = true;
end

%% Reset
if reset
    E_f     = E;
    theta_f = wrapToPiLocal(theta);
    Vg_f    = Vg;
    P_f     = Pg;
    Q_f     = Qg;

    E0_z     = E;
    theta0_z = wrapToPiLocal(theta);
    Vg0_z    = Vg;
    P0_z     = Pg;
    Q0_z     = Qg;

    stableCount = 0;
    locked_z    = false;
    prevSteady  = false;
end

%% 保存上一时刻滤波值，用于计算变化速率
E_prev     = E_f;
theta_prev = theta_f;
Vg_prev    = Vg_f;
P_prev     = P_f;
Q_prev     = Q_f;

%% 递推平均滤波
if enable
    E_f  = (1-alpha)*E_f  + alpha*E;
    Vg_f = (1-alpha)*Vg_f + alpha*Vg;
    P_f  = (1-alpha)*P_f  + alpha*Pg;
    Q_f  = (1-alpha)*Q_f  + alpha*Qg;

    % 角度不能直接普通平均，否则在 +/-pi 附近可能发生跳变。
    % 先计算最短角度差，再递推更新。
    dtheta = wrapToPiLocal(theta - theta_f);
    theta_f = wrapToPiLocal(theta_f + alpha*dtheta);
end

%% 计算滤波量变化速率
rE = abs(E_f - E_prev)/Ts;

dtheta_f = wrapToPiLocal(theta_f - theta_prev);
rTheta = abs(dtheta_f)/Ts;

rVg = abs(Vg_f - Vg_prev)/Ts;
rP  = abs(P_f  - P_prev)/Ts;
rQ  = abs(Q_f  - Q_prev)/Ts;

%% 稳态判据
stableNow = ...
       (rE     <= rE_max)     && ...
       (rTheta <= rTheta_max) && ...
       (rVg    <= rVg_max)    && ...
       (rP     <= rP_max)     && ...
       (rQ     <= rQ_max);

%% 连续稳态计数
if enable && stableNow
    if stableCount < Nhold
        stableCount = stableCount + 1;
    end
else
    stableCount = 0;
end

steady = (stableCount >= Nhold);

%% 工作点锁存
if steady
    if updateMode < 0.5
        % 模式0：
        % 第一次达到稳态后锁存，以后保持不变
        if ~locked_z
            E0_z     = E_f;
            theta0_z = theta_f;
            Vg0_z    = Vg_f;
            P0_z     = P_f;
            Q0_z     = Q_f;
            locked_z = true;
        end

    else
        % 模式1：
        % 只在“非稳态 -> 稳态”的上升沿重新锁存，
        % 避免稳态期间工作点一直追踪当前量。
        if ~prevSteady
            E0_z     = E_f;
            theta0_z = theta_f;
            Vg0_z    = Vg_f;
            P0_z     = P_f;
            Q0_z     = Q_f;
            locked_z = true;
        end
    end
end

prevSteady = steady;

%% 输出
E0     = E0_z;
theta0 = theta0_z;
Vg0    = Vg0_z;
Pg0    = P0_z;
Qg0    = Q0_z;

locked = locked_z;

Ebar     = E_f;
thetabar = theta_f;
Vgbar    = Vg_f;
Pgbar    = P_f;
Qgbar    = Q_f;

end


%% ============================================================
% 局部角度限制函数
% 将角度限制到 [-pi, pi)
%% ============================================================
function y = wrapToPiLocal(x)

y = mod(x + pi, 2*pi) - pi;

end

== matlab function GFMUPS100k_CPP/VSG_Control/无功控制环1/MATLAB Function ==
  data: Vgd input; Eff output; Vgq input; Vsd input; Vsq input; Vg output; Vs output; dU output

function [Eff, Vg, Vs, dU] = fcn(Vgd, Vgq, Vsd, Vsq)
%#codegen
%
% 稳态电压幅值前馈
%
% 输入：
% Vgd, Vgq : 网侧电压dq分量
% Vsd, Vsq : PCC/UPS侧电压dq分量
%
% 输出：
% Eff : 电压幅值前馈补偿量
% Vg  : 网侧电压幅值
% Vs  : PCC侧电压幅值
% dU  : 电压幅值偏差 Vg - Vs

%% 1. 前馈增益
% 初始仿真参数，后续根据结果调整
Kff = 15;

%% 2. 计算dq电压矢量幅值
Vg = sqrt(Vgd*Vgd + Vgq*Vgq);
Vs = sqrt(Vsd*Vsd + Vsq*Vsq);

%% 3. 电压幅值偏差
dU = Vg - Vs;

%% 4. 前馈补偿
Eff = Kff * dU;

end

== matlab function GFMUPS100k_CPP/MATLAB Function2 ==
  data: S_brk input; pref output
function pref = Set_Pref(S_brk)
    % 该函数用于根据并网/离网状态设定 UPS 的有功功率参考值
    % 输入: S_brk (1: 并网, 0: 离网)
    % 输出: pref (有功功率参考值，单位: W)

    if S_brk == 1
        % S_brk = 1 表示并网状态，UPS 待机
        pref = 0;  % 100 kW
    elseif S_brk == 0
        % S_brk = 0 表示离网状态，UPS 满载输出
        pref = 100000; % 100 kW
    else
        % 容错保护：如果 S_brk 信号出现异常，默认保持在较低的安全待机功率
        pref = 10000;  % 100 kW
    end
end

== matlab function GFMUPS100k_CPP/MATLAB Function3 ==
  settings: updateMethod=DISCRETE
  data: v1_pu input; S_grid output; v2_pu input; freq_hz input; d_theta input; d_U input; d_f input; t input; S_brk output; S_sync_ok output; S_sync_en output
function [S_grid, S_brk, S_sync_ok, S_sync_en] = integrated_control(v1_pu, v2_pu, freq_hz, d_theta, d_U, d_f, t)
% 构网型UPS并离网控制综合状态机
% 输入参数:
%   v1_pu, v2_pu, freq_hz - 电网状态检测 (正序pu, 负序pu, 电网频率Hz)
%   d_theta, d_U, d_f     - 预同步检测 (相位差rad, 电压差V, 频率差Hz)
%   t                     - 当前仿真时间 (s)
% 输出参数:
%   S_grid    - 电网状态 (1:正常, 0:故障)
%   S_brk     - 断路器状态 (1:闭合并网, 0:断开离网)
%   S_sync_ok - 预同步完成标志 (1:完成, 0:未完成)
%   S_sync_en - 预同步使能标志 (1:使能, 0:不使能)

    % ==========================================
    % 0. 声明持久化变量 (用于记忆上一时刻的状态和时间)
    % ==========================================
    persistent brk_state;          % 断路器内部状态记忆
    persistent grid_fault_time;    % 记录最近一次电网故障发生的时间点
    persistent sync_start_time;    % 记录预同步条件开始满足的时间点

    % 初始化 (方案 A：系统上电默认离网)
    if isempty(brk_state)
        brk_state = 0;             % 默认离网 (断路器断开)
        grid_fault_time = -1;      % -1 表示当前无故障记录
        sync_start_time = -1;      % -1 表示预同步条件暂未满足
    end

    % ==========================================
    % 1. 电网状态判断 (含 0.1s 故障保持防抖)
    % ==========================================
    V1_MIN = 0.9; V1_MAX = 1.1; V2_MAX = 0.1;
    FREQ_MIN = 49.8; FREQ_MAX = 50.2;
    FAULT_HOLD_TIME = 0.1;         % 故障保持时间 0.1s

    % 实时检测当前电网物理量是否合规
    is_grid_ok_now = (v1_pu >= V1_MIN) && (v1_pu <= V1_MAX) && ...
                     (v2_pu <= V2_MAX) && ...
                     (freq_hz >= FREQ_MIN) && (freq_hz <= FREQ_MAX);

    % 屏蔽仿真前 0.02s 的暂态不准确数据
    if t < 0.2
        is_grid_ok_now = false; 
    end

    % 故障保持逻辑处理
    if ~is_grid_ok_now
        % 只要出现物理量异常，不断刷新故障时间戳，并输出故障状态
        grid_fault_time = t; 
        S_grid = 0;
    else
        % 物理量恢复正常，检查是否度过了 0.1s 的“惩罚期(保持期)”
        if (t - grid_fault_time) < FAULT_HOLD_TIME && grid_fault_time >= 0
            S_grid = 0; % 还在保持期内，强行按故障处理，防止反复跳变
        else
            S_grid = 1; % 彻底恢复正常
        end
    end

    % ==========================================
    % 2. 预同步使能逻辑
    % ==========================================
    % 使用上一时刻的断路器状态 (brk_state) 来判断
    if S_grid == 1 && brk_state == 0
        S_sync_en = 1; % 电网正常且断路器断开，启动预同步
    else
        S_sync_en = 0;
    end

    % ==========================================
    % 3. 预同步条件判断 (含 0.005s 接通延时)
    % ==========================================
    SYNC_DELAY_TIME = 0.005; % 满足条件需持续 0.005s
    S_sync_ok = 0;           % 默认输出为 0

    if S_sync_en == 1
        % 检查三大误差是否进入阈值 (加入 abs 绝对值计算，替代之前的 Simulink 模块)
        is_sync_cond_met = (abs(d_theta) < 0.087266) && ...
                           (abs(d_U) < 15) && ...
                           (abs(d_f) < 0.05);

        if is_sync_cond_met
            if sync_start_time < 0
                % 第一眼看到条件满足，记录当前时间
                sync_start_time = t; 
            elseif (t - sync_start_time) >= SYNC_DELAY_TIME
                % 持续时间达标，发出同步完成信号
                S_sync_ok = 1;       
            end
        else
            % 只要条件一被破坏，立刻重置计时器
            sync_start_time = -1;    
        end
    else
        % 如果未使能预同步，也要重置计时器
        sync_start_time = -1;        
    end

    % ==========================================
    % 4. 断路器状态机更新
    % ==========================================
    if S_grid == 0
        % 第一优先级：电网故障(或处于故障保持期)，强制离网
        brk_state = 0; 
    else
        % 电网处于正常且稳定状态
        if brk_state == 0
            % 当前为离网状态，等待预同步完成
            if S_sync_ok == 1
                brk_state = 1; % 预同步完成，合闸并网！
            end
        else
            % 当前已经并网，锁定状态保持不变
            brk_state = 1; 
        end
    end

    % 赋值输出
    S_brk = brk_state; 
end

== matlab function GFMUPS100k_CPP/基于自适应虚拟电流/自适应PI/adaptive_PI ==
  data: Ivq_re input; Kp_base input; Kp_act output; Ki_base input; Ki_act output
function [Kp_act, Ki_act] = Adaptive_PI_Design(Ivq_re, Kp_base, Ki_base)
    % Adaptive_PI_Design - 基于误差反馈的参数自适应 PI 控制策略
    % 对应论文公式 (5-8) 至 (5-11)
    % 
    % 输入:
    %   Ivq_re:  重构后的虚拟电流幅值 (即论文中的 Ivq')
    %   Kp_base: 比例增益初始基准值 Kp0
    %   Ki_base: 积分增益初始基准值 Ki0
    
    % --- 1. 物理参数定义与量纲统一 ---
    W_base = 314.16;         % 基准角频率 (100*pi rad/s)
    Limit_Physical = 34.97; % 允许的最大角频率补偿量上限 (rad/s)
    
    % 将物理极限量转换为标幺值 (p.u.)，确保与 Kp_base 量纲一致
    % dw_max 对应论文中的 \Delta\omega_{max}
    dw_max = Limit_Physical / W_base; 
    
    % --- 2. 计算形状因子 \mu ---
    % 对应论文公式 (5-10): \mu = (K_{p0} / \Delta\omega_{max})^2
    mu = (Kp_base / dw_max)^2;
    
    % --- 3. 计算自适应衰减因子 \eta ---
    % 对应论文公式 (5-8): \eta = 1 / \sqrt{1 + \mu * (Ivq')^2}
    % 该连续函数自带小误差下的全增益特性，无需分段阈值
    eta = 1 / sqrt(1 + mu * (Ivq_re^2));
    
    % --- 4. 输出最终控制增益 ---
    % (a) 比例增益：对应公式 (5-11)，保证大误差下的频率安全性
    Kp_act = Kp_base * eta;
    
    % (b) 积分增益：引入 \eta 的三次方衰减，对应文稿防积分饱和逻辑
    Ki_act = Ki_base * (eta^3); 
    
end

== matlab function GFMUPS100k_CPP/基于自适应虚拟电流/重构 ==
  data: Ivd input; Ivq input; Ivq_re output; Iv input
function Ivq_re = Geo_Reconstruction(Ivd, Ivq, Iv)
% Geometric Modulus Reconstruction (弦长几何重构)
% Inputs (必须是标幺值!):
%   Ivd:  d轴虚拟电流 (范围 approx -2.0 ~ 2.0 p.u.)
%   Ivq:  q轴虚拟电流 (范围 approx -2.0 ~ 2.0 p.u.)
%   Iv:   虚拟电流幅值 (通常为 1.0 ~ 2.0 p.u.)
% Output:
%   Ivq_re: 重构后的标幺化弦长误差，送入自适应 PI 控制器

    %% 1. 方向判断
    % 使用 q 轴分量符号判断超前/滞后
    direction = sign(Ivq);
    
    % 处理零点奇异性 (虽然浮点数很难正好撞上0)
    if direction == 0
        direction = 1; 
    end
    
    %% 2. 几何模值计算 (Chord Length Calculation)
    % 计算从当前矢量 (Ivd, Ivq) 到目标矢量 (Iv, 0) 的欧氏距离
    % 物理含义：这是拉动系统同步的“最大几何张力”
    
    term1 = (Ivd - Iv)^2;
    term2 = Ivq^2;
    Error_geo = sqrt(term1 + term2);
    
    %% 3. 信号重构
    % 输出带符号的弦长误差
    Ivq_re = direction * Error_geo;
    
end

== matlab function GFMUPS100k_CPP/SVPWM调制/SVPWM/大扇区 ==
  data: u input; N output; theta output
function [N,theta] = BigVector(u)
N=0;
theta=0;
thetaset=ceil(u*3/pi);
u1=u;
u2=u-pi/3;
u3=u-2*pi/3;
u4=u-pi;
u5=u-4*pi/3;
u6=u-5*pi/3;
if(thetaset==1)
    theta=u1;
    N=4;
end
if(thetaset==2)
    theta=u2;
    N=5;
end
if(thetaset==3)
    theta=u3;
    N=6;
end
if(thetaset==4)
    theta=u4;
    N=1;
end
if(thetaset==5)
    theta=u5;
    N=2;
end
if(thetaset==6)
    theta=u6;
    N=3;
end

== matlab function GFMUPS100k_CPP/A practical and fast sequence components detection scheme for three-phase unbalanced grid voltage.2021/Subsystem1/MATLAB Function1 ==
  settings: updateMethod=DISCRETE
  data: u input; y_out output
function y_out = maf_filter(u)
    % 滑动平均滤波法 (MAF)
    % 采样时间: 1e-4 s, 电网基波频率: 50 Hz
    % 窗口长度 L: T/2 = 0.01 s -> 100 个采样点 (用于消除 3, 5, 7 次等奇次谐波)
    
    % 定义持久化变量
    persistent buf_maf sum_maf idx_maf
    
    if isempty(buf_maf)
        buf_maf = zeros(100, 1);
        sum_maf = 0;
        idx_maf = 1;
    end
    
    % 读取窗口中最旧的值，即公式 (41) 中的 u(t - L*DeltaT)
    u_old = buf_maf(idx_maf);
    
    % 采用递推方式更新滑动窗口的总和，大幅降低每步运算量
    sum_maf = sum_maf + u - u_old; 
    
    % 计算当前步的平均值
    y_out = sum_maf / 100;
    
    % 更新环形缓冲区
    buf_maf(idx_maf) = u;
    
    % 更新索引
    idx_maf = idx_maf + 1;
    if idx_maf > 100
        idx_maf = 1;
    end
end

== matlab function GFMUPS100k_CPP/A practical and fast sequence components detection scheme for three-phase unbalanced grid voltage.2021/T1\T2矩阵变换 ==
  data: U_alpha input; U_pos output; U_beta input; U_neg output
function [U_pos, U_neg] = Sequence_Extraction(U_alpha, U_beta)
% 输入:
%   U_alpha: 3x1 向量，[ua; ub; uc] (实际采样值)
%   U_beta:  3x1 向量，[ua_beta; ub_beta; uc_beta] (STD模块计算值)
% 输出:
%   U_pos: 3x1 向量，三相正序电压瞬时值
%   U_neg: 3x1 向量，三相负序电压瞬时值

% 定义矩阵 T1_alpha 和 T1_beta (论文公式 10)
T1_alpha = (1/6) * [2 -1 -1; -1 2 -1; -1 -1 2];
T1_beta  = (sqrt(3)/6) * [0 -1 1; 1 0 -1; -1 1 0];

% 定义矩阵 T2_alpha 和 T2_beta (论文公式 11)
% T2_alpha 通常等于 T1_alpha
% T2_beta 通常等于 -T1_beta
T2_alpha = T1_alpha;
T2_beta  = -T1_beta;

% 计算正序分量 U+ = T1a*Ua + T1b*Ub
U_pos = T1_alpha * U_alpha + T1_beta * U_beta;

% 计算负序分量 U- = T2a*Ua + T2b*Ub
U_neg = T2_alpha * U_alpha + T2_beta * U_beta;

end

== matlab function GFMUPS100k_CPP/A practical and fast sequence components detection scheme for three-phase unbalanced grid voltage.2021/Ubeta计算/MATLAB Function10 ==
  data: u_alpha input; u_beta output; Ts input; omega input; N input
function u_beta = MultiPoint_OSG(u_alpha, Ts, omega, N)
% MULTIPOINT_OSG: 基于多点最小二乘最优拟合的正交信号构造
% 
% 参数说明:
%   u_alpha : 当前时刻的单相采样输入 u(k)
%   Ts      : 采样周期 (例如 1e-4)
%   omega   : 电网基波角频率 (例如 2*pi*50)
%   N       : 拟合使用的总点数 (建议值：4 代表4点拟合；21 代表2毫秒全密集拟合)

% 声明持久变量：历史缓冲区、常数系数数组、初始化标志
persistent u_buffer C_coeffs initialized;

% 初始化模块 (仅在系统启动的第一个采样周期执行一次，极大节省算力)
if isempty(initialized)
    % 1. 计算相邻采样点的电角度步长
    alpha = omega * Ts;
    
    % 2. 预生成约束矩阵的三角函数项
    c = zeros(N, 1);
    s = zeros(N, 1);
    for i = 1:N
        c(i) = cos((i-1) * alpha);
        s(i) = sin((i-1) * alpha);
    end
    
    % 3. 计算中间常数矩阵
    M11 = sum(c.^2);
    M12 = sum(c .* s);
    M22 = sum(s.^2);
    Delta = M11 * M22 - M12^2;
    
    % 4. 计算最优抗噪系数 C0, C1 ... C_N-1
    C_coeffs = zeros(N, 1);
    for i = 1:N
        C_coeffs(i) = (M12 * c(i) - M11 * s(i)) / Delta;
    end
    
    % 【极性匹配说明】
    % 您原先的代码 u_beta = (u(k-1) - u(k)*cos)/sin 
    % 在输入为 sin(wt) 时，输出的是 -cos(wt)。
    % 为了确保替换后系统后续的 PLL 或控制逻辑不受极性翻转的影响，这里乘以 -1。
    C_coeffs = -C_coeffs; 
    
    % 5. 初始化历史数据移位寄存器 (全 0)
    u_buffer = zeros(N, 1);
    initialized = true;
end

% ================= 实 时 运 行 区 =================

% 1. 更新历史数据缓冲区 (FIFO 移位)
% 将旧数据向后平移，新数据 u_alpha 推入头部 (u_buffer(1) 代表当前 k 时刻)
for i = N:-1:2
    u_buffer(i) = u_buffer(i-1);
end
u_buffer(1) = u_alpha;

% 2. 核心正交计算 (向量内积乘加运算)
% 等效于: u_beta = C0*u(k) + C1*u(k-1) + C2*u(k-2) + ...
u_beta = sum(C_coeffs .* u_buffer);

end

== matlab function GFMUPS100k_CPP/A practical and fast sequence components detection scheme for three-phase unbalanced grid voltage.2021/Ubeta计算/MATLAB Function11 ==
  data: u_alpha input; u_beta output; Ts input; omega input; N input
function u_beta = MultiPoint_OSG(u_alpha, Ts, omega, N)
% MULTIPOINT_OSG: 基于多点最小二乘最优拟合的正交信号构造
% 
% 参数说明:
%   u_alpha : 当前时刻的单相采样输入 u(k)
%   Ts      : 采样周期 (例如 1e-4)
%   omega   : 电网基波角频率 (例如 2*pi*50)
%   N       : 拟合使用的总点数 (建议值：4 代表4点拟合；21 代表2毫秒全密集拟合)

% 声明持久变量：历史缓冲区、常数系数数组、初始化标志
persistent u_buffer C_coeffs initialized;

% 初始化模块 (仅在系统启动的第一个采样周期执行一次，极大节省算力)
if isempty(initialized)
    % 1. 计算相邻采样点的电角度步长
    alpha = omega * Ts;
    
    % 2. 预生成约束矩阵的三角函数项
    c = zeros(N, 1);
    s = zeros(N, 1);
    for i = 1:N
        c(i) = cos((i-1) * alpha);
        s(i) = sin((i-1) * alpha);
    end
    
    % 3. 计算中间常数矩阵
    M11 = sum(c.^2);
    M12 = sum(c .* s);
    M22 = sum(s.^2);
    Delta = M11 * M22 - M12^2;
    
    % 4. 计算最优抗噪系数 C0, C1 ... C_N-1
    C_coeffs = zeros(N, 1);
    for i = 1:N
        C_coeffs(i) = (M12 * c(i) - M11 * s(i)) / Delta;
    end
    
    % 【极性匹配说明】
    % 您原先的代码 u_beta = (u(k-1) - u(k)*cos)/sin 
    % 在输入为 sin(wt) 时，输出的是 -cos(wt)。
    % 为了确保替换后系统后续的 PLL 或控制逻辑不受极性翻转的影响，这里乘以 -1。
    C_coeffs = -C_coeffs; 
    
    % 5. 初始化历史数据移位寄存器 (全 0)
    u_buffer = zeros(N, 1);
    initialized = true;
end

% ================= 实 时 运 行 区 =================

% 1. 更新历史数据缓冲区 (FIFO 移位)
% 将旧数据向后平移，新数据 u_alpha 推入头部 (u_buffer(1) 代表当前 k 时刻)
for i = N:-1:2
    u_buffer(i) = u_buffer(i-1);
end
u_buffer(1) = u_alpha;

% 2. 核心正交计算 (向量内积乘加运算)
% 等效于: u_beta = C0*u(k) + C1*u(k-1) + C2*u(k-2) + ...
u_beta = sum(C_coeffs .* u_buffer);

end
